simulink model "Particle_swarm_based_PV_MPPT"  (R2017a)
settings: Solver=ode45  StartTime=0.0  StopTime=1  RelTol=1e-3  EnableMultiTasking=on
undefined symbols (not defined in the file): dEgdT, EgRef, gcbh, k1, Rsh_array5pc, sigbuilder_block, sps_rtmsupport, Tref_K, Ts, VT_ref
libraries: powerlib x16, spsPVarrayModel x3, simulink x1, powerlib_meascontrol x1
(part 6 of 6)

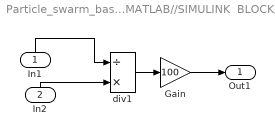
== system Particle_swarm_based_PV_MPPT/MATLAB//SIMULINK  BLOCK/      ==
  In1 : Inport
  In2 : Inport  Port=2
  Gain : Gain  Gain=100
  div1 : Product  Inputs=/*  RndMeth=Zero
  Out1 : Outport
  wires:
  Gain/1 -> Out1/1
  div1/1 -> Gain/1
  In2/1 -> div1/2
  In1/1 -> div1/1

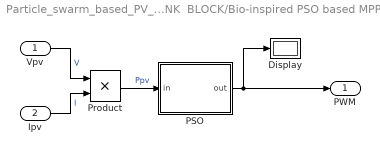
== system Particle_swarm_based_PV_MPPT/MATLAB//SIMULINK  BLOCK/Bio-inspired PSO based MPPT ==
  Vpv : Inport
  Ipv : Inport  Port=2
  Display : Display
  PSO : MATLAB Function  TreatAsAtomicUnit=on  SystemSampleTime=Ts
  Product : Product
  PWM : Outport
  wires:
  Product/1 -> PSO/1(in)  "Ppv"
  Ipv/1 -> Product/2  "I"
  Vpv/1 -> Product/1  "V"
  PSO/1(out) -> Display/1, PWM/1

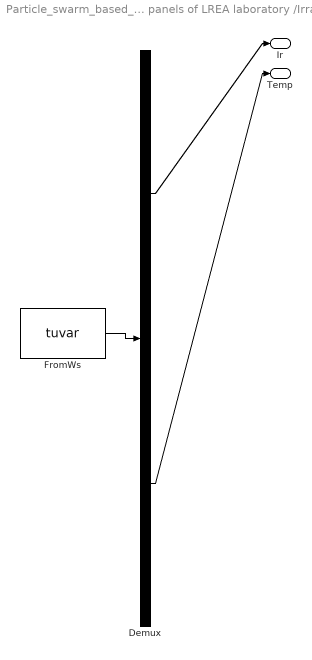
== system Particle_swarm_based_PV_MPPT/MATLAB//SIMULINK  BLOCK/	PV panels of LREA laboratory /Irradiance  ==
  Demux : Demux  Tag=STV Demux  Outputs=2
  FromWs : FromWorkspace  Tag=STV FromWs  VariableName=tuvar  SampleTime=0
      SigBuilderData=|
      | common.afterFinalStr = 'Extrapolate'
      | common.sampleTime = '0'
      | dataSet(1).timeRange = [0 2]
      | dataSet(1).name = 'Constant Irradiance'
      | dataSet(2).timeRange = [0 2]
      | dataSet(2).name = 'Step Irradiance'
      | dataSet(3).timeRange = [0 1]
      | dataSet(3).name = 'Ramp-up/down Irradiance'
      | sbobj.Groups(1).Name = 'Constant Irradiance'
      | sbobj.Groups(1).Signals(1).Name = 'Ir'
      | sbobj.Groups(1).Signals(1).XData = [0 2]
      | sbobj.Groups(1).Signals(1).YData = [1000 1000]
      | sbobj.Groups(1).Signals(2).Name = 'Temp'
      | sbobj.Groups(1).Signals(2).XData = [0 1 1 2]
      | sbobj.Groups(1).Signals(2).YData = [0 0 1 1]
      | sbobj.Groups(1).TimeRange = [0 2]
      | sbobj.Groups(2).Name = 'Step Irradiance'
      | sbobj.Groups(2).Signals(1).Name = 'Ir'
      | sbobj.Groups(2).Signals(1).XData = [0 0.252 0.252 2]
      | sbobj.Groups(2).Signals(1).YData = [600 600 1000 1000]
      | sbobj.Groups(2).Signals(2).Name = 'Temp'
      | sbobj.Groups(2).Signals(2).XData = [0 1 1 2]
      | sbobj.Groups(2).Signals(2).YData = [0 0 1 1]
      | sbobj.Groups(2).TimeRange = [0 2]
      | sbobj.Groups(3).Name = 'Ramp-up/down Irradiance'
      | sbobj.Groups(3).Signals(1).Name = 'Ir'
      | sbobj.Groups(3).Signals(1).XData = [0 0.3 0.3 0.4 0.4 0.5 0.5 1]
      | sbobj.Groups(3).Signals(1).YData = [1000 1000 800 795 600 600 400 395]
      | sbobj.Groups(3).Signals(2).Name = 'Temp'
      | sbobj.Groups(3).Signals(2).XData = [0 1]
      | sbobj.Groups(3).Signals(2).YData = [25 25]
      | sbobj.Groups(3).TimeRange = [0 1]
  Ir : Outport  Tag=STV Outport
  Temp : Outport  Tag=STV Outport  Port=2
  wires:
  Demux/1 -> Ir/1
  FromWs/1 -> Demux/1
  Demux/2 -> Temp/1

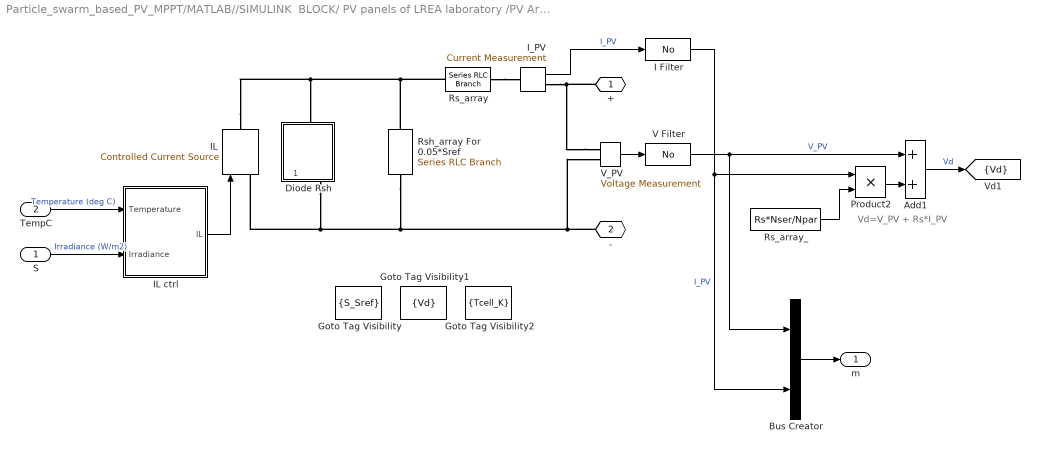
== system Particle_swarm_based_PV_MPPT/MATLAB//SIMULINK  BLOCK/	PV panels of LREA laboratory /PV Array ==
  note: Vd=V_PV + Rs*I_PV
  S : Inport
  TempC : Inport  Port=2
  Add1 : Sum
  Bus Creator : BusCreator  Inputs=2
  Diode Rsh : Subsystem
      mask Display:
      | plot(-75,-50,100,150, [-15 -15 43 -15 -15 -75],[50 8 50 92 50 50], ...
      |     [43 43],[8 94],[100 43], [50 50])
  Goto Tag Visibility : GotoTagVisibility  GotoTag=S_Sref
  Goto Tag Visibility1 : GotoTagVisibility  GotoTag=Vd
  Goto Tag Visibility2 : GotoTagVisibility  GotoTag=Tcell_K
  I Filter : spsPVarrayModel/No  VariantControl=Variant1
  IL : powerlib/Electrical Sources/Controlled Current Source  Initialize=on  Source_Type=AC  Amplitude=0  Phase=0  Frequency=0  Measurements=None
  IL ctrl : Subsystem
  I_PV : powerlib/Measurements/Current Measurement  PhasorSimulation=off  OutputType=Complex  PSBequivalent=0
  Product2 : Product  Inputs=**  RndMeth=Zero
  Rs_array : powerlib/Elements/Series RLC Branch  LConnTagsString=__new0  RConnTagsString=__new0  BranchType=R  Resistance=Rs*Nser/Npar  Inductance=1e-3  SetiL0=off  InitialCurrent=0  Capacitance=1e-6  Setx0=off  InitialVoltage=0  Measurements=None
  Rs_array_ : Constant  Value=Rs*Nser/Npar
  Rsh_array For 0.05*Sref : powerlib/Elements/Series RLC Branch  LConnTagsString=__new0  RConnTagsString=__new0  BranchType=R  Resistance=Rsh_array5pc  Inductance=1e-3  SetiL0=off  InitialCurrent=0  Capacitance=1e-6  Setx0=off  InitialVoltage=0  Measurements=None
  V Filter : spsPVarrayModel/No  VariantControl=Variant1
  V_PV : powerlib/Measurements/Voltage Measurement  PhasorSimulation=off  OutputType=Complex  PSBequivalent=0
  + : PMIOPort  Port=1  Side=Right
  - : PMIOPort  Port=2  Side=Right
  m : Outport
  tag scope: Vd=scoped
  wires:
  V Filter/1 -> Add1/1, Bus Creator/1  "V_PV"
  I Filter/1 -> Product2/1, Bus Creator/2  "I_PV"
  V_PV/1 -> V Filter/1
  IL ctrl/1(IL) -> IL/1
  Bus Creator/1 -> m/1
  Rs_array_/1 -> Product2/2
  Product2/1 -> Add1/2
  I_PV/1 -> I Filter/1  "I_PV"
  Add1/1 -> [Vd]  "Vd"
  S/1 -> IL ctrl/2(Irradiance)  "Irradiance (W/m2)"
  TempC/1 -> IL ctrl/1(Temperature)  "Temperature (deg C)"
  connections:
  Rs_array/RConn1 -- I_PV/LConn1
  IL/LConn1 -- Diode Rsh/RConn1 -- Rsh_array For 0.05*Sref/RConn1 -- -/RConn1 -- V_PV/LConn2
  IL/RConn1 -- Rsh_array For 0.05*Sref/LConn1 -- Rs_array/LConn1 -- Diode Rsh/LConn1
  V_PV/LConn1 -- I_PV/RConn1 -- +/RConn1

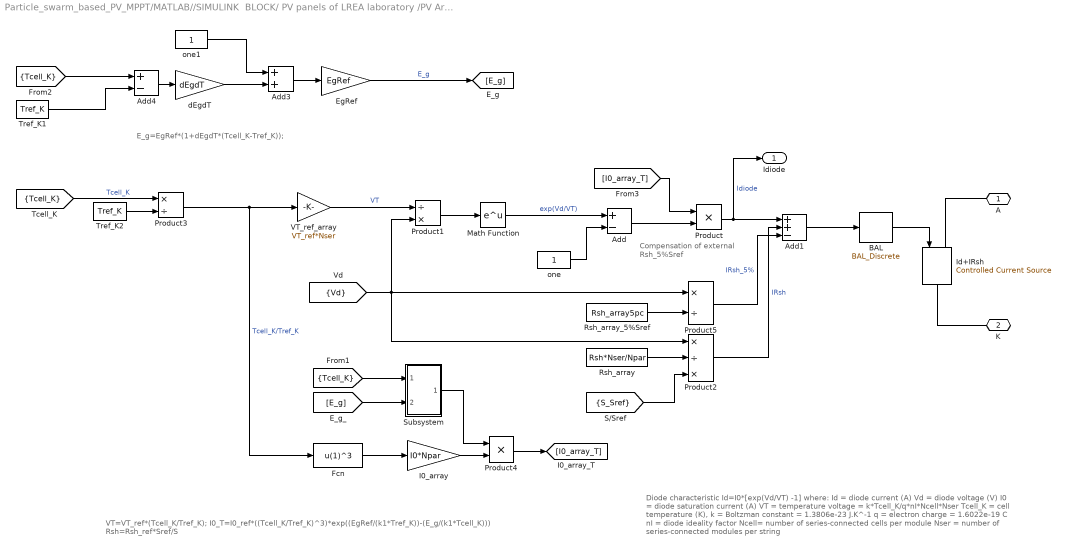
== system Particle_swarm_based_PV_MPPT/MATLAB//SIMULINK  BLOCK/	PV panels of LREA laboratory /PV Array/Diode Rsh ==
  note: Compensation of
      | external Rsh_5%Sref
  note: Diode characteristic
      |    Id=I0*[exp(Vd/VT) -1]
      |
      | where:
      |      Id = diode current (A)
      |      Vd = diode voltage (V)
      |      I0 = diode saturation current (A)
      |      VT = temperature voltage = k*Tcell_K/q*nI*Ncell*Nser
      | Tcell_K = cell temperature (K),
      |       k = Boltzman constant = 1.3806e-23 J.K^-1
      |       q = electron charge = 1.6022e-19 C
      |      nI = diode ideality factor
      |    Ncell= number of series-connected cells per module
      |    Nser = number of series-connected modules per string
  note: VT=VT_ref*(Tcell_K/Tref_K);
      | I0_T=I0_ref*((Tcell_K/Tref_K)^3)*exp((EgRef/(k1*Tref_K))-(E_g/(k1*Tcell_K)))
      | Rsh=Rsh_ref*Sref/S
  note: E_g=EgRef*(1+dEgdT*(Tcell_K-Tref_K));
  Add : Sum  Inputs=+-
  Add1 : Sum  Inputs=++-
  Add3 : Sum
  Add4 : Sum  Inputs=+-
  BAL : spsPVarrayModel/BAL_Discrete  VariantControl=NoBAL
  EgRef : Gain  Gain=EgRef
  Fcn : Fcn  Expr=u(1)^3
  I0_array : Gain  Gain=I0*Npar
  Id+IRsh : powerlib/Electrical Sources/Controlled Current Source  Initialize=on  Source_Type=AC  Amplitude=0  Phase=0  Frequency=0  Measurements=None
  Math Function : Math  SaturateOnIntegerOverflow=on
  Product : Product  RndMeth=Zero
  Product1 : Product  Inputs=/*  RndMeth=Zero
  Product2 : Product  Inputs=*/*  RndMeth=Zero
  Product3 : Product  Inputs=*/  RndMeth=Zero
  Product4 : Product  Inputs=**  RndMeth=Zero
  Product5 : Product  Inputs=*/  RndMeth=Zero
  Rsh_array : Constant  Value=Rsh*Nser/Npar
  Rsh_array_5%Sref : Constant  Value=Rsh_array5pc
  Subsystem : Subsystem
  Tref_K1 : Constant  Value=Tref_K
  Tref_K2 : Constant  Value=Tref_K
  VT_ref_array : Gain  Gain=VT_ref*Nser
  dEgdT : Gain  Gain=dEgdT
  one : Constant
  one1 : Constant
  A : PMIOPort  Port=1  Side=Left
  K : PMIOPort  Port=2  Side=Right
  Idiode : Outport
  wires:
  BAL/1 -> Id+IRsh/1
  Add1/1 -> BAL/1
  Product5/1 -> Add1/3  "IRsh_5%"
  Rsh_array_5%Sref/1 -> Product5/2
  Math Function/1 -> Add/1  "exp(Vd/VT)"
  Product2/1 -> Add1/2  "IRsh"
  Product/1 -> Add1/1, Idiode/1  "Idiode"
  Product1/1 -> Math Function/1
  one/1 -> Add/2
  Rsh_array/1 -> Product2/2
  [Tcell_K] -> Product3/1  "Tcell_K"
  Product3/1 -> VT_ref_array/1, Fcn/1  "Tcell_K/Tref_K"
  one1/1 -> Add3/1
  Add4/1 -> dEgdT/1
  dEgdT/1 -> Add3/2
  Add3/1 -> EgRef/1
  EgRef/1 -> [E_g]  "E_g"
  I0_array/1 -> Product4/2
  Fcn/1 -> I0_array/1
  [Tcell_K] -> Add4/1
  Tref_K1/1 -> Add4/2
  Subsystem/1(exp) -> Product4/1
  [Tcell_K] -> Subsystem/1(Tcell_K)
  [E_g] -> Subsystem/2(E_g)
  Tref_K2/1 -> Product3/2
  Product4/1 -> [I0_array_T]
  Add/1 -> Product/2
  VT_ref_array/1 -> Product1/1  "VT"
  [I0_array_T] -> Product/1
  [S_Sref] -> Product2/3
  [Vd] -> Product5/1, Product2/1, Product1/2
  connections:
  Id+IRsh/RConn1 -- K/RConn1
  A/RConn1 -- Id+IRsh/LConn1

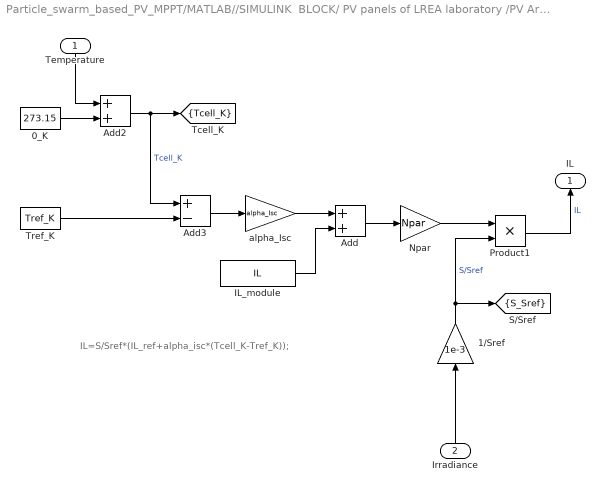
== system Particle_swarm_based_PV_MPPT/MATLAB//SIMULINK  BLOCK/	PV panels of LREA laboratory /PV Array/IL ctrl ==
  note: IL=S/Sref*(IL_ref+alpha_isc*(Tcell_K-Tref_K));
  Temperature : Inport
  Irradiance : Inport  Port=2
  0_K : Constant  Value=273.15
  1/Sref : Gain  Gain=1e-3
  Add : Sum
  Add2 : Sum
  Add3 : Sum  Inputs=+-
  IL_module : Constant  Value=IL
  Npar : Gain  Gain=Npar
  Product1 : Product  Inputs=**  RndMeth=Zero
  Tref_K : Constant  Value=Tref_K
  alpha_Isc : Gain  Gain=alpha_Isc
  IL : Outport
  tag scope: S_Sref=scoped, Tcell_K=scoped
  wires:
  Temperature/1 -> Add2/1
  Irradiance/1 -> 1/Sref/1
  alpha_Isc/1 -> Add/1
  Add3/1 -> alpha_Isc/1
  Tref_K/1 -> Add3/2
  Product1/1 -> IL/1  "IL"
  IL_module/1 -> Add/2
  0_K/1 -> Add2/2
  Add/1 -> Npar/1
  Add2/1 -> Add3/1, [Tcell_K]  "Tcell_K"
  Npar/1 -> Product1/1
  1/Sref/1 -> Product1/2, [S_Sref]  "S/Sref"

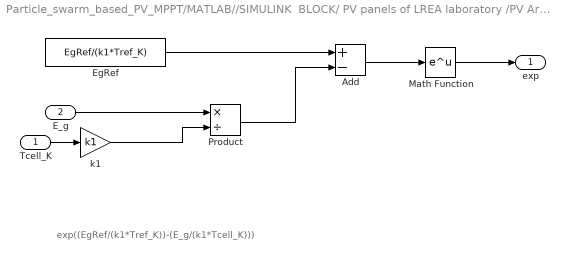
== system Particle_swarm_based_PV_MPPT/MATLAB//SIMULINK  BLOCK/	PV panels of LREA laboratory /PV Array/Diode Rsh/Subsystem ==
  note: exp((EgRef/(k1*Tref_K))-(E_g/(k1*Tcell_K)))
  Tcell_K : Inport
  E_g : Inport  Port=2
  Add : Sum  Inputs=+-
  EgRef : Constant  Value=EgRef/(k1*Tref_K)
  Math Function : Math  SaturateOnIntegerOverflow=on
  Product : Product  Inputs=*/
  k1 : Gain  Gain=k1
  exp : Outport
  wires:
  EgRef/1 -> Add/1
  E_g/1 -> Product/1
  Tcell_K/1 -> k1/1
  k1/1 -> Product/2
  Product/1 -> Add/2
  Add/1 -> Math Function/1
  Math Function/1 -> exp/1

== matlab function Particle_swarm_based_PV_MPPT/MATLAB//SIMULINK  BLOCK/Bio-inspired PSO based MPPT/PSO ==
  data: out output; in input
function out=PSO(in)
%% PSO Specification
w=0.01;
c1=0.8;
c2=0.8;
N=8;
pmin=0.1;
pmax=0.9;


%% Starting Up
persistent p;
if isempty(p) 
    %Create empty particle
    p.x = linspace(pmin,pmax,N);
    p.v = zeros(1,N);
    p.y = zeros(1,N);
	p.bx = zeros(1,N);
    p.by = zeros(1,N);
    p.bg=pmin;
    p.k=1;
    out=p.x(p.k);
else


%% Input
p.y(p.k)=in;


%% Best Particle
if p.y(p.k)>p.by(p.k)
    p.bx(p.k)=p.x(p.k);
    p.by(p.k)=p.y(p.k);
end


%% PSO Algorithm
p.v(p.k)=w*p.v(p.k)+c1*(p.bx(p.k)-p.x(p.k))+c2*(p.bg-p.x(p.k));
p.x(p.k)=p.x(p.k)+p.v(p.k);


%% Limit Position
if p.x(p.k)<=pmin
   p.x(p.k)=pmin;
end
if p.x(p.k)>=pmax
    p.x(p.k)=pmax;
end


%% Update Particle Turn,k
p.k=p.k+1;
if p.k>N
    [a,b]=max(p.by);
    p.bg=p.bx(b);
    p.k=1;
end


%% Output
out=p.x(p.k);


end


%% About
% Razman Ayop
% Created on 31 October 2019
